simulink model "Platoon_Year1_CACC_fixed"  (R2026a)
settings: Solver=ode23tb  StopTime=inf  MaxStep=0.01  RelTol=1e-4  AbsTol=1e-6
values from neighbouring files (symbols this model uses):
  Cyber_AttackType = 0    [init_platoon_params.m]
  Cyber_FDI_Bias = 2    [init_platoon_params.m]
  Cyber_FDI_Field = 3    [init_platoon_params.m]
  Cyber_ReplayDelay = 0.5    [init_platoon_params.m]
  Cyber_ResidualThreshold = 1.0    (= 1)    [init_platoon_params.m]
  Cyber_TargetVehicle = 1    [init_platoon_params.m]
  D_DES = 10    [init_platoon_params.m]    (also in platoon_cyber_ui.m = evalin('base','D_DES'))
  h_CTH = 0.6    [init_platoon_params.m]
  Kd_CACC = 0.7    [init_platoon_params.m]
  Kd_PD = 0.10    (= 0.1)    [init_platoon_params.m]
  KP_CACC = 0.2    [init_platoon_params.m]
  Kp_PD = 0.8    [init_platoon_params.m]
  L_VEH = 4    [init_platoon_params.m]    (also in platoon_cyber_ui.m = evalin('base','L_VEH'))
  v0 = 0    [init_platoon_params.m]
  x0_f = x0_leader - (1:4) * gap0    [init_platoon_params.m]
  x0_leader = 130    [init_platoon_params.m]
undefined symbols (not defined in the file or in its folder): t_step
libraries: simulink x4
settings Model: Creator=robert  LastModifiedBy=Robert

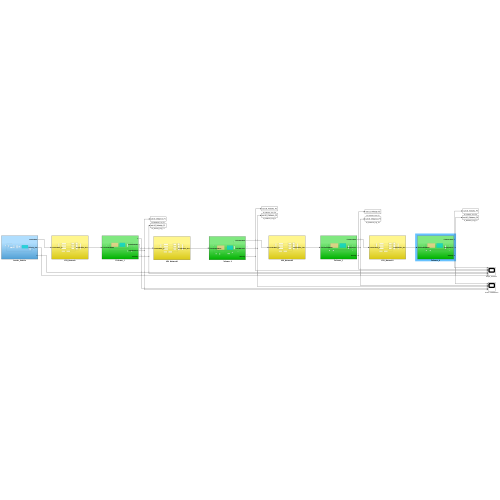
[thumbnail: Simulink's stored preview of the top-level diagram]
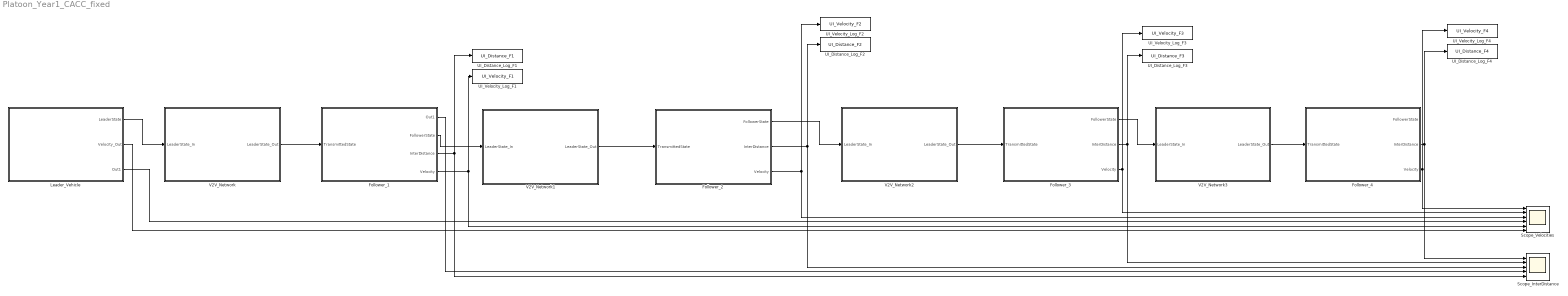
== system Platoon_Year1_CACC_fixed ==
  Follower_1 : Subsystem
  Follower_2 : Subsystem
  Follower_3 : Subsystem
  Follower_4 : Subsystem
  Leader_Vehicle : Subsystem
  Scope_InterDistance : Scope  NumInputPorts=5
      settings: ActiveDisplayYMinimum=-70.886144233669683  ActiveDisplayYMaximum=99.147830095673541
  Scope_Velocities : Scope  NumInputPorts=6
      settings: ActiveDisplayYMinimum=-4.6500669764690308  ActiveDisplayYMaximum=39.524777851018328
  UI_Distance_Log_F1 : ToWorkspace  VariableName=UI_Distance_F1  SaveFormat=Timeseries  SampleTime=-1
  UI_Distance_Log_F2 : ToWorkspace  VariableName=UI_Distance_F2  SaveFormat=Timeseries  SampleTime=-1
  UI_Distance_Log_F3 : ToWorkspace  VariableName=UI_Distance_F3  SaveFormat=Timeseries  SampleTime=-1
  UI_Distance_Log_F4 : ToWorkspace  VariableName=UI_Distance_F4  SaveFormat=Timeseries  SampleTime=-1
  UI_Velocity_Log_F1 : ToWorkspace  VariableName=UI_Velocity_F1  SaveFormat=Timeseries  SampleTime=-1
  UI_Velocity_Log_F2 : ToWorkspace  VariableName=UI_Velocity_F2  SaveFormat=Timeseries  SampleTime=-1
  UI_Velocity_Log_F3 : ToWorkspace  VariableName=UI_Velocity_F3  SaveFormat=Timeseries  SampleTime=-1
  UI_Velocity_Log_F4 : ToWorkspace  VariableName=UI_Velocity_F4  SaveFormat=Timeseries  SampleTime=-1
  V2V_Network : Subsystem
  V2V_Network1 : Subsystem
  V2V_Network2 : Subsystem
  V2V_Network3 : Subsystem
  wires:
  Follower_3/1(FollowerState) -> V2V_Network3/1(LeaderState_In)
  Follower_2/1(FollowerState) -> V2V_Network2/1(LeaderState_In)
  Follower_1/2(FollowerState) -> V2V_Network1/1(LeaderState_In)
  V2V_Network1/1(LeaderState_Out) -> Follower_2/1(TransmittedState)
  V2V_Network2/1(LeaderState_Out) -> Follower_3/1(TransmittedState)
  V2V_Network3/1(LeaderState_Out) -> Follower_4/1(TransmittedState)
  Leader_Vehicle/1(LeaderState) -> V2V_Network/1(LeaderState_In)
  V2V_Network/1(LeaderState_Out) -> Follower_1/1(TransmittedState)
  Leader_Vehicle/2(Velocity_Out) -> Scope_Velocities/6
  Follower_1/4(Velocity) -> Scope_Velocities/5, UI_Velocity_Log_F1/1
  Follower_2/3(Velocity) -> UI_Velocity_Log_F2/1, Scope_Velocities/3
  Follower_3/3(Velocity) -> Scope_Velocities/2, UI_Velocity_Log_F3/1
  Follower_4/3(Velocity) -> Scope_Velocities/1, UI_Velocity_Log_F4/1
  Follower_4/2(InterDistance) -> Scope_InterDistance/1, UI_Distance_Log_F4/1
  Follower_3/2(InterDistance) -> Scope_InterDistance/2, UI_Distance_Log_F3/1
  Follower_2/2(InterDistance) -> UI_Distance_Log_F2/1, Scope_InterDistance/3
  Follower_1/3(InterDistance) -> Scope_InterDistance/5, UI_Distance_Log_F1/1
  Follower_1/1(Out1) -> Scope_InterDistance/4
  Leader_Vehicle/3(Out1) -> Scope_Velocities/4

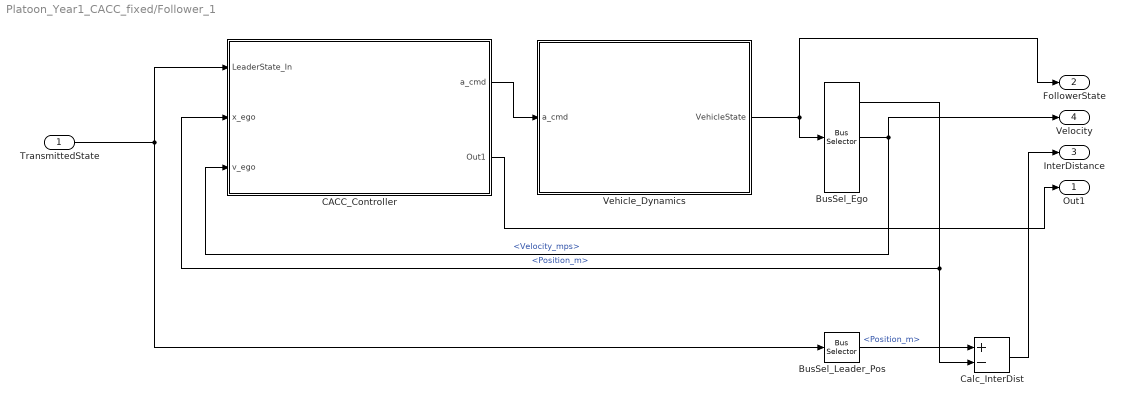
== system Platoon_Year1_CACC_fixed/Follower_1 ==
  TransmittedState : Inport
  BusSel_Ego : BusSelector  OutputSignals=Position_m,Velocity_mps,Accel_mps2
  BusSel_Leader_Pos : BusSelector  OutputSignals=Position_m
  CACC_Controller : Subsystem  TreatAsAtomicUnit=on
  Calc_InterDist : Sum  Inputs=+-
  Vehicle_Dynamics : Subsystem  TreatAsAtomicUnit=on
  Out1 : Outport
  FollowerState : Outport  Port=2
  InterDistance : Outport  Port=3
  Velocity : Outport  Port=4
  wires:
  TransmittedState/1 -> CACC_Controller/1(LeaderState_In), BusSel_Leader_Pos/1
  CACC_Controller/1(a_cmd) -> Vehicle_Dynamics/1(a_cmd)
  Vehicle_Dynamics/1(VehicleState) -> BusSel_Ego/1, FollowerState/1
  BusSel_Ego/1 -> CACC_Controller/2(x_ego), Calc_InterDist/2  "<Position_m>"
  BusSel_Ego/2 -> Velocity/1, CACC_Controller/3(v_ego)  "<Velocity_mps>"
  BusSel_Leader_Pos/1 -> Calc_InterDist/1  "<Position_m>"
  Calc_InterDist/1 -> InterDistance/1
  CACC_Controller/2(Out1) -> Out1/1

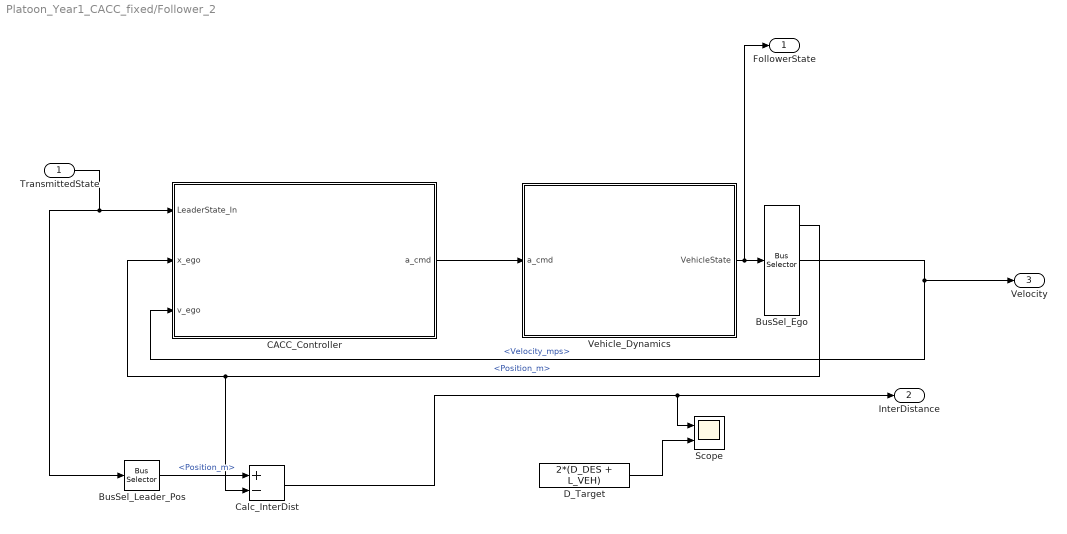
== system Platoon_Year1_CACC_fixed/Follower_2 ==
  TransmittedState : Inport
  BusSel_Ego : BusSelector  OutputSignals=Position_m,Velocity_mps,Accel_mps2
  BusSel_Leader_Pos : BusSelector  OutputSignals=Position_m
  CACC_Controller : Subsystem  TreatAsAtomicUnit=on
  Calc_InterDist : Sum  Inputs=+-
  D_Target : Constant  Value=2*(D_DES + L_VEH)
  Scope : Scope  NumInputPorts=2
      settings: ActiveDisplayYMinimum=-29.731224200783366  ActiveDisplayYMaximum=61.45407779195633
  Vehicle_Dynamics : Subsystem  TreatAsAtomicUnit=on
  FollowerState : Outport
  InterDistance : Outport  Port=2
  Velocity : Outport  Port=3
  wires:
  TransmittedState/1 -> CACC_Controller/1(LeaderState_In), BusSel_Leader_Pos/1
  CACC_Controller/1(a_cmd) -> Vehicle_Dynamics/1(a_cmd)
  Vehicle_Dynamics/1(VehicleState) -> BusSel_Ego/1, FollowerState/1
  BusSel_Ego/1 -> CACC_Controller/2(x_ego), Calc_InterDist/2  "<Position_m>"
  BusSel_Ego/2 -> CACC_Controller/3(v_ego), Velocity/1  "<Velocity_mps>"
  BusSel_Leader_Pos/1 -> Calc_InterDist/1  "<Position_m>"
  Calc_InterDist/1 -> InterDistance/1, Scope/1
  D_Target/1 -> Scope/2

== system Platoon_Year1_CACC_fixed/Follower_3 ==
  TransmittedState : Inport
  BusSel_Ego : BusSelector  OutputSignals=Position_m,Velocity_mps,Accel_mps2
  BusSel_Leader_Pos : BusSelector  OutputSignals=Position_m
  CACC_Controller : Subsystem  TreatAsAtomicUnit=on
  Calc_InterDist : Sum  Inputs=+-
  Vehicle_Dynamics : Subsystem  TreatAsAtomicUnit=on
  FollowerState : Outport
  InterDistance : Outport  Port=2
  Velocity : Outport  Port=3
  wires:
  TransmittedState/1 -> CACC_Controller/1(LeaderState_In), BusSel_Leader_Pos/1
  CACC_Controller/1(a_cmd) -> Vehicle_Dynamics/1(a_cmd)
  Vehicle_Dynamics/1(VehicleState) -> BusSel_Ego/1, FollowerState/1
  BusSel_Ego/1 -> CACC_Controller/2(x_ego), Calc_InterDist/2  "<Position_m>"
  BusSel_Ego/2 -> CACC_Controller/3(v_ego), Velocity/1  "<Velocity_mps>"
  BusSel_Leader_Pos/1 -> Calc_InterDist/1  "<Position_m>"
  Calc_InterDist/1 -> InterDistance/1

== system Platoon_Year1_CACC_fixed/Follower_4 ==
  TransmittedState : Inport
  BusSel_Ego : BusSelector  OutputSignals=Position_m,Velocity_mps,Accel_mps2
  BusSel_Leader_Pos : BusSelector  OutputSignals=Position_m
  CACC_Controller : Subsystem  TreatAsAtomicUnit=on
  Calc_InterDist : Sum  Inputs=+-
  Vehicle_Dynamics : Subsystem  TreatAsAtomicUnit=on
  FollowerState : Outport
  InterDistance : Outport  Port=2
  Velocity : Outport  Port=3
  wires:
  TransmittedState/1 -> CACC_Controller/1(LeaderState_In), BusSel_Leader_Pos/1
  CACC_Controller/1(a_cmd) -> Vehicle_Dynamics/1(a_cmd)
  Vehicle_Dynamics/1(VehicleState) -> BusSel_Ego/1, FollowerState/1
  BusSel_Ego/1 -> CACC_Controller/2(x_ego), Calc_InterDist/2  "<Position_m>"
  BusSel_Ego/2 -> CACC_Controller/3(v_ego), Velocity/1  "<Velocity_mps>"
  BusSel_Leader_Pos/1 -> Calc_InterDist/1  "<Position_m>"
  Calc_InterDist/1 -> InterDistance/1

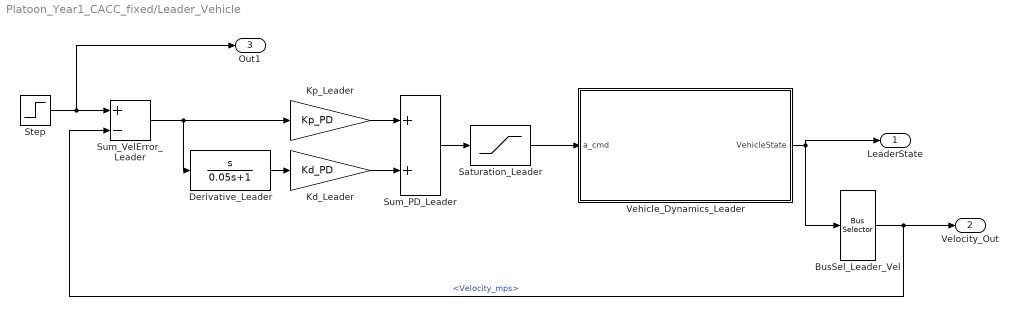
== system Platoon_Year1_CACC_fixed/Leader_Vehicle ==
  BusSel_Leader_Vel : BusSelector  OutputSignals=Velocity_mps
  Derivative_Leader : TransferFcn  Numerator=[1 0]  Denominator=[0.05 1]
  Kd_Leader : Gain  Gain=Kd_PD
  Kp_Leader : Gain  Gain=Kp_PD
  Saturation_Leader : Saturate  UpperLimit=2  LowerLimit=-4
  Step : Step  Time=t_step  InitialValue=v0  FinalValue=v_cmd_final  SampleTime=0.01
  Sum_PD_Leader : Sum
  Sum_VelError_Leader : Sum  Inputs=+-
  Vehicle_Dynamics_Leader : Subsystem  TreatAsAtomicUnit=on
  LeaderState : Outport
  Velocity_Out : Outport  Port=2
  Out1 : Outport  Port=3
  wires:
  Step/1 -> Out1/1, Sum_VelError_Leader/1
  Sum_VelError_Leader/1 -> Kp_Leader/1, Derivative_Leader/1
  Derivative_Leader/1 -> Kd_Leader/1
  Sum_PD_Leader/1 -> Saturation_Leader/1
  Saturation_Leader/1 -> Vehicle_Dynamics_Leader/1(a_cmd)
  Vehicle_Dynamics_Leader/1(VehicleState) -> LeaderState/1, BusSel_Leader_Vel/1
  BusSel_Leader_Vel/1 -> Sum_VelError_Leader/2, Velocity_Out/1  "<Velocity_mps>"
  Kd_Leader/1 -> Sum_PD_Leader/2
  Kp_Leader/1 -> Sum_PD_Leader/1

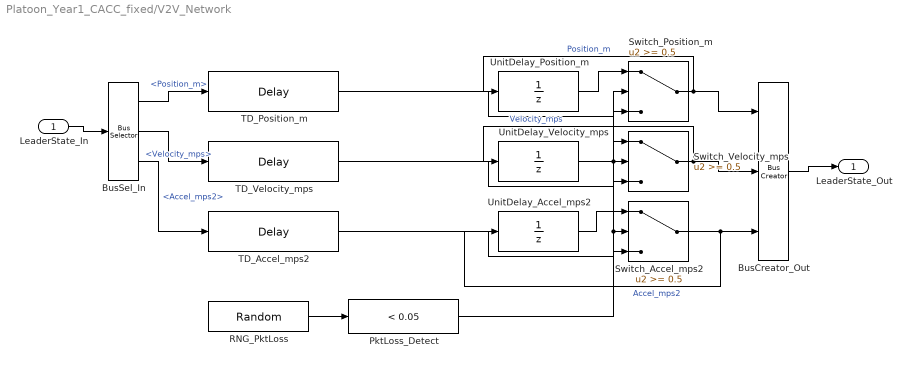
== system Platoon_Year1_CACC_fixed/V2V_Network ==
  LeaderState_In : Inport
  BusCreator_Out : BusCreator  Inputs=3
  BusSel_In : BusSelector  OutputSignals=Position_m,Velocity_mps,Accel_mps2
  PktLoss_Detect : simulink/Logic and Bit Operations/Compare To Constant  relop=<  const=0.05  OutDataTypeStr=boolean
  RNG_PktLoss : UniformRandomNumber  Minimum=0  Seed=42  SampleTime=0.01
  Switch_Accel_mps2 : Switch  Threshold=0.5  SaturateOnIntegerOverflow=off  InputSameDT=off
  Switch_Position_m : Switch  Threshold=0.5  SaturateOnIntegerOverflow=off  InputSameDT=off
  Switch_Velocity_mps : Switch  Threshold=0.5  SaturateOnIntegerOverflow=off  InputSameDT=off
  TD_Accel_mps2 : TransportDelay  DelayTime=0.02
  TD_Position_m : TransportDelay  DelayTime=0.02  InitialOutput=x0_leader
  TD_Velocity_mps : TransportDelay  DelayTime=0.02  InitialOutput=v0
  UnitDelay_Accel_mps2 : UnitDelay  SampleTime=0.01
  UnitDelay_Position_m : UnitDelay  InitialCondition=x0_leader  SampleTime=0.01
  UnitDelay_Velocity_mps : UnitDelay  InitialCondition=v0  SampleTime=0.01
  LeaderState_Out : Outport
  wires:
  BusSel_In/1 -> TD_Position_m/1  "<Position_m>"
  BusSel_In/2 -> TD_Velocity_mps/1  "<Velocity_mps>"
  BusSel_In/3 -> TD_Accel_mps2/1  "<Accel_mps2>"
  RNG_PktLoss/1 -> PktLoss_Detect/1
  UnitDelay_Position_m/1 -> Switch_Position_m/1
  PktLoss_Detect/1 -> Switch_Position_m/2, Switch_Velocity_mps/2, Switch_Accel_mps2/2
  TD_Position_m/1 -> Switch_Position_m/3
  Switch_Position_m/1 -> UnitDelay_Position_m/1, BusCreator_Out/1  "Position_m"
  UnitDelay_Velocity_mps/1 -> Switch_Velocity_mps/1
  TD_Velocity_mps/1 -> Switch_Velocity_mps/3
  Switch_Velocity_mps/1 -> UnitDelay_Velocity_mps/1, BusCreator_Out/2  "Velocity_mps"
  UnitDelay_Accel_mps2/1 -> Switch_Accel_mps2/1
  TD_Accel_mps2/1 -> Switch_Accel_mps2/3
  Switch_Accel_mps2/1 -> UnitDelay_Accel_mps2/1, BusCreator_Out/3  "Accel_mps2"
  BusCreator_Out/1 -> LeaderState_Out/1
  LeaderState_In/1 -> BusSel_In/1

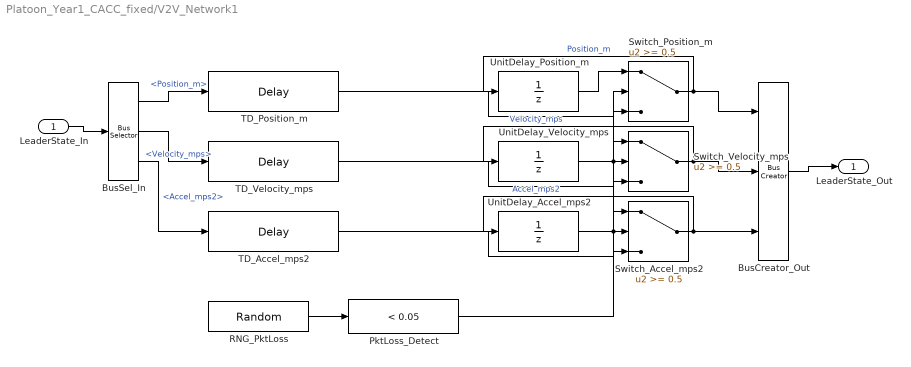
== system Platoon_Year1_CACC_fixed/V2V_Network1 ==
  LeaderState_In : Inport
  BusCreator_Out : BusCreator  Inputs=3
  BusSel_In : BusSelector  OutputSignals=Position_m,Velocity_mps,Accel_mps2
  PktLoss_Detect : simulink/Logic and Bit Operations/Compare To Constant  relop=<  const=0.05  OutDataTypeStr=boolean
  RNG_PktLoss : UniformRandomNumber  Minimum=0  Seed=137  SampleTime=0.01
  Switch_Accel_mps2 : Switch  Threshold=0.5  SaturateOnIntegerOverflow=off  InputSameDT=off
  Switch_Position_m : Switch  Threshold=0.5  SaturateOnIntegerOverflow=off  InputSameDT=off
  Switch_Velocity_mps : Switch  Threshold=0.5  SaturateOnIntegerOverflow=off  InputSameDT=off
  TD_Accel_mps2 : TransportDelay  DelayTime=0.02
  TD_Position_m : TransportDelay  DelayTime=0.02  InitialOutput=x0_f(1)
  TD_Velocity_mps : TransportDelay  DelayTime=0.02  InitialOutput=v0
  UnitDelay_Accel_mps2 : UnitDelay  SampleTime=0.01
  UnitDelay_Position_m : UnitDelay  InitialCondition=x0_f(1)  SampleTime=0.01
  UnitDelay_Velocity_mps : UnitDelay  InitialCondition=v0  SampleTime=0.01
  LeaderState_Out : Outport
  wires:
  BusSel_In/1 -> TD_Position_m/1  "<Position_m>"
  BusSel_In/2 -> TD_Velocity_mps/1  "<Velocity_mps>"
  BusSel_In/3 -> TD_Accel_mps2/1  "<Accel_mps2>"
  RNG_PktLoss/1 -> PktLoss_Detect/1
  UnitDelay_Position_m/1 -> Switch_Position_m/1
  PktLoss_Detect/1 -> Switch_Position_m/2, Switch_Velocity_mps/2, Switch_Accel_mps2/2
  TD_Position_m/1 -> Switch_Position_m/3
  Switch_Position_m/1 -> UnitDelay_Position_m/1, BusCreator_Out/1  "Position_m"
  UnitDelay_Velocity_mps/1 -> Switch_Velocity_mps/1
  TD_Velocity_mps/1 -> Switch_Velocity_mps/3
  Switch_Velocity_mps/1 -> UnitDelay_Velocity_mps/1, BusCreator_Out/2  "Velocity_mps"
  UnitDelay_Accel_mps2/1 -> Switch_Accel_mps2/1
  TD_Accel_mps2/1 -> Switch_Accel_mps2/3
  Switch_Accel_mps2/1 -> UnitDelay_Accel_mps2/1, BusCreator_Out/3  "Accel_mps2"
  BusCreator_Out/1 -> LeaderState_Out/1
  LeaderState_In/1 -> BusSel_In/1

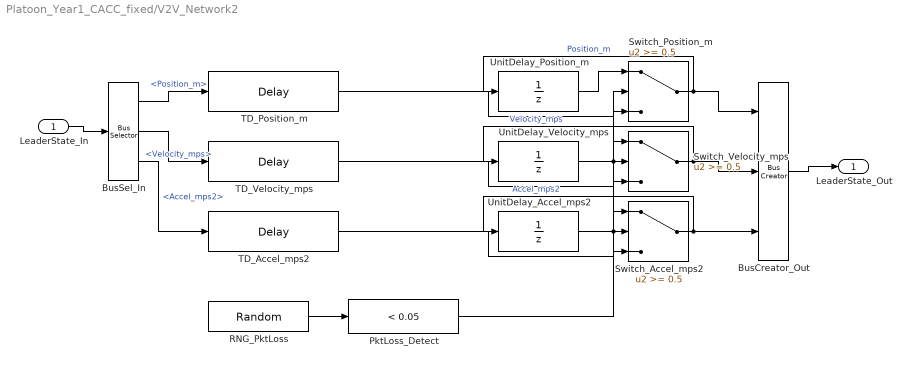
== system Platoon_Year1_CACC_fixed/V2V_Network2 ==
  LeaderState_In : Inport
  BusCreator_Out : BusCreator  Inputs=3
  BusSel_In : BusSelector  OutputSignals=Position_m,Velocity_mps,Accel_mps2
  PktLoss_Detect : simulink/Logic and Bit Operations/Compare To Constant  relop=<  const=0.05  OutDataTypeStr=boolean
  RNG_PktLoss : UniformRandomNumber  Minimum=0  Seed=251  SampleTime=0.01
  Switch_Accel_mps2 : Switch  Threshold=0.5  SaturateOnIntegerOverflow=off  InputSameDT=off
  Switch_Position_m : Switch  Threshold=0.5  SaturateOnIntegerOverflow=off  InputSameDT=off
  Switch_Velocity_mps : Switch  Threshold=0.5  SaturateOnIntegerOverflow=off  InputSameDT=off
  TD_Accel_mps2 : TransportDelay  DelayTime=0.02
  TD_Position_m : TransportDelay  DelayTime=0.02  InitialOutput=x0_f(2)
  TD_Velocity_mps : TransportDelay  DelayTime=0.02  InitialOutput=v0
  UnitDelay_Accel_mps2 : UnitDelay  SampleTime=0.01
  UnitDelay_Position_m : UnitDelay  InitialCondition=x0_f(2)  SampleTime=0.01
  UnitDelay_Velocity_mps : UnitDelay  InitialCondition=v0  SampleTime=0.01
  LeaderState_Out : Outport
  wires:
  BusSel_In/1 -> TD_Position_m/1  "<Position_m>"
  BusSel_In/2 -> TD_Velocity_mps/1  "<Velocity_mps>"
  BusSel_In/3 -> TD_Accel_mps2/1  "<Accel_mps2>"
  RNG_PktLoss/1 -> PktLoss_Detect/1
  UnitDelay_Position_m/1 -> Switch_Position_m/1
  PktLoss_Detect/1 -> Switch_Position_m/2, Switch_Velocity_mps/2, Switch_Accel_mps2/2
  TD_Position_m/1 -> Switch_Position_m/3
  Switch_Position_m/1 -> UnitDelay_Position_m/1, BusCreator_Out/1  "Position_m"
  UnitDelay_Velocity_mps/1 -> Switch_Velocity_mps/1
  TD_Velocity_mps/1 -> Switch_Velocity_mps/3
  Switch_Velocity_mps/1 -> UnitDelay_Velocity_mps/1, BusCreator_Out/2  "Velocity_mps"
  UnitDelay_Accel_mps2/1 -> Switch_Accel_mps2/1
  TD_Accel_mps2/1 -> Switch_Accel_mps2/3
  Switch_Accel_mps2/1 -> UnitDelay_Accel_mps2/1, BusCreator_Out/3  "Accel_mps2"
  BusCreator_Out/1 -> LeaderState_Out/1
  LeaderState_In/1 -> BusSel_In/1

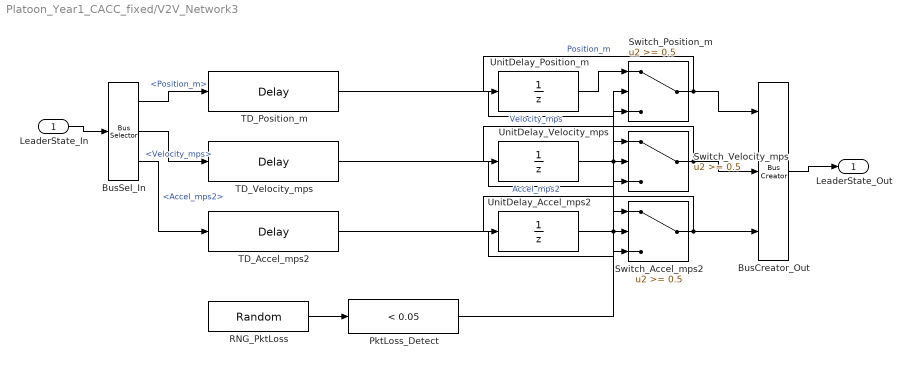
== system Platoon_Year1_CACC_fixed/V2V_Network3 ==
  LeaderState_In : Inport
  BusCreator_Out : BusCreator  Inputs=3
  BusSel_In : BusSelector  OutputSignals=Position_m,Velocity_mps,Accel_mps2
  PktLoss_Detect : simulink/Logic and Bit Operations/Compare To Constant  relop=<  const=0.05  OutDataTypeStr=boolean
  RNG_PktLoss : UniformRandomNumber  Minimum=0  Seed=389  SampleTime=0.01
  Switch_Accel_mps2 : Switch  Threshold=0.5  SaturateOnIntegerOverflow=off  InputSameDT=off
  Switch_Position_m : Switch  Threshold=0.5  SaturateOnIntegerOverflow=off  InputSameDT=off
  Switch_Velocity_mps : Switch  Threshold=0.5  SaturateOnIntegerOverflow=off  InputSameDT=off
  TD_Accel_mps2 : TransportDelay  DelayTime=0.02
  TD_Position_m : TransportDelay  DelayTime=0.02  InitialOutput=x0_f(3)
  TD_Velocity_mps : TransportDelay  DelayTime=0.02  InitialOutput=v0
  UnitDelay_Accel_mps2 : UnitDelay  SampleTime=0.01
  UnitDelay_Position_m : UnitDelay  InitialCondition=x0_f(3)  SampleTime=0.01
  UnitDelay_Velocity_mps : UnitDelay  InitialCondition=v0  SampleTime=0.01
  LeaderState_Out : Outport
  wires:
  BusSel_In/1 -> TD_Position_m/1  "<Position_m>"
  BusSel_In/2 -> TD_Velocity_mps/1  "<Velocity_mps>"
  BusSel_In/3 -> TD_Accel_mps2/1  "<Accel_mps2>"
  RNG_PktLoss/1 -> PktLoss_Detect/1
  UnitDelay_Position_m/1 -> Switch_Position_m/1
  PktLoss_Detect/1 -> Switch_Position_m/2, Switch_Velocity_mps/2, Switch_Accel_mps2/2
  TD_Position_m/1 -> Switch_Position_m/3
  Switch_Position_m/1 -> UnitDelay_Position_m/1, BusCreator_Out/1  "Position_m"
  UnitDelay_Velocity_mps/1 -> Switch_Velocity_mps/1
  TD_Velocity_mps/1 -> Switch_Velocity_mps/3
  Switch_Velocity_mps/1 -> UnitDelay_Velocity_mps/1, BusCreator_Out/2  "Velocity_mps"
  UnitDelay_Accel_mps2/1 -> Switch_Accel_mps2/1
  TD_Accel_mps2/1 -> Switch_Accel_mps2/3
  Switch_Accel_mps2/1 -> UnitDelay_Accel_mps2/1, BusCreator_Out/3  "Accel_mps2"
  BusCreator_Out/1 -> LeaderState_Out/1
  LeaderState_In/1 -> BusSel_In/1

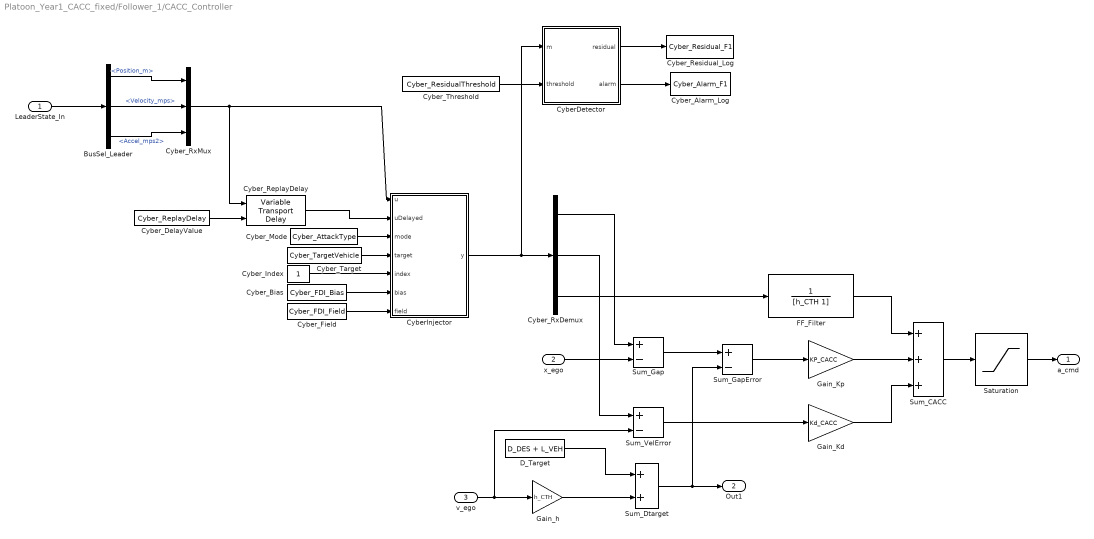
== system Platoon_Year1_CACC_fixed/Follower_1/CACC_Controller ==
  LeaderState_In : Inport
  x_ego : Inport  Port=2
  v_ego : Inport  Port=3
  BusSel_Leader : BusSelector  OutputSignals=Position_m,Velocity_mps,Accel_mps2
  CyberDetector : MATLAB Function  TreatAsAtomicUnit=on
  CyberInjector : MATLAB Function  TreatAsAtomicUnit=on
  Cyber_Alarm_Log : ToWorkspace  VariableName=Cyber_Alarm_F1  SaveFormat=Timeseries  SampleTime=-1
  Cyber_Bias : Constant  Value=Cyber_FDI_Bias
  Cyber_DelayValue : Constant  Value=Cyber_ReplayDelay
  Cyber_Field : Constant  Value=Cyber_FDI_Field
  Cyber_Index : Constant
  Cyber_Mode : Constant  Value=Cyber_AttackType
  Cyber_ReplayDelay : VariableTransportDelay  MaximumDelay=5  InitialOutput=[x0_leader; v0; 0]  MaximumPoints=8192
  Cyber_Residual_Log : ToWorkspace  VariableName=Cyber_Residual_F1  SaveFormat=Timeseries  SampleTime=-1
  Cyber_RxDemux : Demux  Outputs=3
  Cyber_RxMux : Mux  Inputs=3
  Cyber_Target : Constant  Value=Cyber_TargetVehicle
  Cyber_Threshold : Constant  Value=Cyber_ResidualThreshold
  D_Target : Constant  Value=D_DES + L_VEH
  FF_Filter : TransferFcn  Denominator=[h_CTH 1]
  Gain_Kd : Gain  Gain=Kd_CACC
  Gain_Kp : Gain  Gain=KP_CACC
  Gain_h : Gain  Gain=h_CTH
  Saturation : Saturate  UpperLimit=2  LowerLimit=-4
  Sum_CACC : Sum  Inputs=+++
  Sum_Dtarget : Sum
  Sum_Gap : Sum  Inputs=+-
  Sum_GapError : Sum  Inputs=+-
  Sum_VelError : Sum  Inputs=+-
  a_cmd : Outport
  Out1 : Outport  Port=2
  wires:
  BusSel_Leader/3 -> Cyber_RxMux/3  "<Accel_mps2>"
  CyberDetector/2(alarm) -> Cyber_Alarm_Log/1
  LeaderState_In/1 -> BusSel_Leader/1
  BusSel_Leader/1 -> Cyber_RxMux/1  "<Position_m>"
  Cyber_DelayValue/1 -> Cyber_ReplayDelay/2
  Cyber_RxMux/1 -> CyberInjector/1(u), Cyber_ReplayDelay/1
  Sum_GapError/1 -> Gain_Kp/1
  BusSel_Leader/2 -> Cyber_RxMux/2  "<Velocity_mps>"
  Sum_CACC/1 -> Saturation/1
  Cyber_ReplayDelay/1 -> CyberInjector/2(uDelayed)
  Cyber_Mode/1 -> CyberInjector/3(mode)
  Cyber_Target/1 -> CyberInjector/4(target)
  Gain_Kp/1 -> Sum_CACC/2
  Cyber_Index/1 -> CyberInjector/5(index)
  Cyber_Bias/1 -> CyberInjector/6(bias)
  Cyber_Field/1 -> CyberInjector/7(field)
  CyberInjector/1(y) -> Cyber_RxDemux/1, CyberDetector/1(m)
  Cyber_Threshold/1 -> CyberDetector/2(threshold)
  v_ego/1 -> Sum_VelError/2, Gain_h/1
  CyberDetector/1(residual) -> Cyber_Residual_Log/1
  Cyber_RxDemux/1 -> Sum_Gap/1
  Cyber_RxDemux/2 -> Sum_VelError/1
  Cyber_RxDemux/3 -> FF_Filter/1
  x_ego/1 -> Sum_Gap/2
  D_Target/1 -> Sum_Dtarget/1
  Gain_h/1 -> Sum_Dtarget/2
  Sum_Gap/1 -> Sum_GapError/1
  Sum_VelError/1 -> Gain_Kd/1
  Sum_Dtarget/1 -> Out1/1, Sum_GapError/2
  FF_Filter/1 -> Sum_CACC/1
  Gain_Kd/1 -> Sum_CACC/3
  Saturation/1 -> a_cmd/1

== system Platoon_Year1_CACC_fixed/Follower_1/Vehicle_Dynamics ==
  a_cmd : Inport
  BusCreator_VehState : BusCreator  Inputs=3
  Engine_Lag_TF : TransferFcn  Denominator=[0.15 1]
  Int_a2v : Integrator  InitialCondition=v0
  Int_v2x : Integrator  InitialCondition=104
  VehicleState : Outport
  wires:
  a_cmd/1 -> Engine_Lag_TF/1
  Engine_Lag_TF/1 -> Int_a2v/1, BusCreator_VehState/3  "Accel_mps2"
  Int_a2v/1 -> Int_v2x/1, BusCreator_VehState/2  "Velocity_mps"
  Int_v2x/1 -> BusCreator_VehState/1  "Position_m"
  BusCreator_VehState/1 -> VehicleState/1

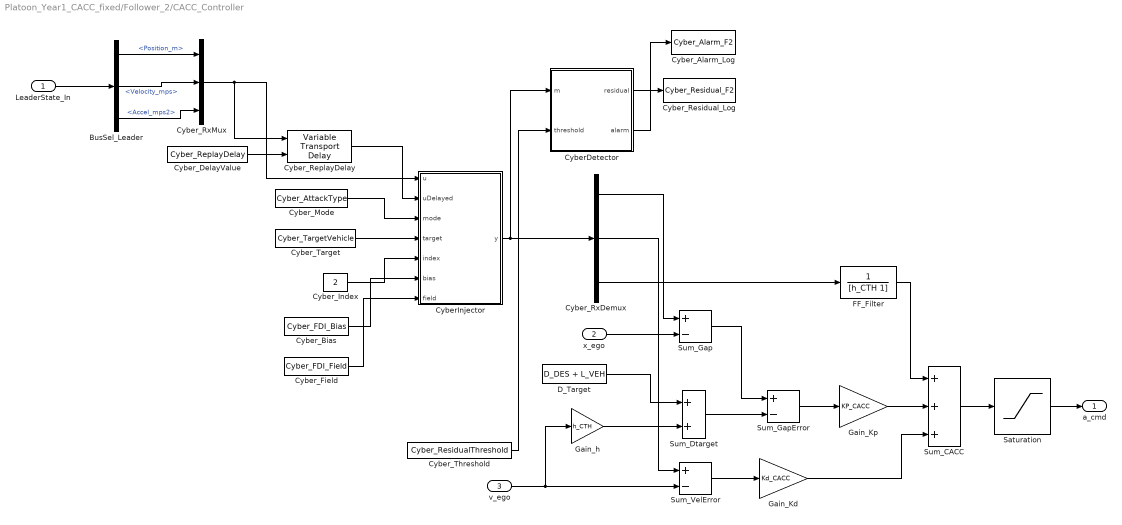
== system Platoon_Year1_CACC_fixed/Follower_2/CACC_Controller ==
  LeaderState_In : Inport
  x_ego : Inport  Port=2
  v_ego : Inport  Port=3
  BusSel_Leader : BusSelector  OutputSignals=Position_m,Velocity_mps,Accel_mps2
  CyberDetector : MATLAB Function  TreatAsAtomicUnit=on
  CyberInjector : MATLAB Function  TreatAsAtomicUnit=on
  Cyber_Alarm_Log : ToWorkspace  VariableName=Cyber_Alarm_F2  SaveFormat=Timeseries  SampleTime=-1
  Cyber_Bias : Constant  Value=Cyber_FDI_Bias
  Cyber_DelayValue : Constant  Value=Cyber_ReplayDelay
  Cyber_Field : Constant  Value=Cyber_FDI_Field
  Cyber_Index : Constant  Value=2
  Cyber_Mode : Constant  Value=Cyber_AttackType
  Cyber_ReplayDelay : VariableTransportDelay  MaximumDelay=5  InitialOutput=[x0_f(1); v0; 0]  MaximumPoints=8192
  Cyber_Residual_Log : ToWorkspace  VariableName=Cyber_Residual_F2  SaveFormat=Timeseries  SampleTime=-1
  Cyber_RxDemux : Demux  Outputs=3
  Cyber_RxMux : Mux  Inputs=3
  Cyber_Target : Constant  Value=Cyber_TargetVehicle
  Cyber_Threshold : Constant  Value=Cyber_ResidualThreshold
  D_Target : Constant  Value=D_DES + L_VEH
  FF_Filter : TransferFcn  Denominator=[h_CTH 1]
  Gain_Kd : Gain  Gain=Kd_CACC
  Gain_Kp : Gain  Gain=KP_CACC
  Gain_h : Gain  Gain=h_CTH
  Saturation : Saturate  UpperLimit=2  LowerLimit=-4
  Sum_CACC : Sum  Inputs=+++
  Sum_Dtarget : Sum
  Sum_Gap : Sum  Inputs=+-
  Sum_GapError : Sum  Inputs=+-
  Sum_VelError : Sum  Inputs=+-
  a_cmd : Outport
  wires:
  LeaderState_In/1 -> BusSel_Leader/1
  BusSel_Leader/2 -> Cyber_RxMux/2  "<Velocity_mps>"
  BusSel_Leader/1 -> Cyber_RxMux/1  "<Position_m>"
  BusSel_Leader/3 -> Cyber_RxMux/3  "<Accel_mps2>"
  FF_Filter/1 -> Sum_CACC/1
  Cyber_RxMux/1 -> CyberInjector/1(u), Cyber_ReplayDelay/1
  Cyber_Bias/1 -> CyberInjector/6(bias)
  Cyber_Mode/1 -> CyberInjector/3(mode)
  Cyber_RxDemux/2 -> Sum_VelError/1
  Cyber_DelayValue/1 -> Cyber_ReplayDelay/2
  Gain_Kp/1 -> Sum_CACC/2
  Cyber_ReplayDelay/1 -> CyberInjector/2(uDelayed)
  Cyber_Target/1 -> CyberInjector/4(target)
  Cyber_Index/1 -> CyberInjector/5(index)
  Cyber_Field/1 -> CyberInjector/7(field)
  x_ego/1 -> Sum_Gap/2
  CyberInjector/1(y) -> Cyber_RxDemux/1, CyberDetector/1(m)
  Cyber_Threshold/1 -> CyberDetector/2(threshold)
  v_ego/1 -> Sum_VelError/2, Gain_h/1
  CyberDetector/1(residual) -> Cyber_Residual_Log/1
  Gain_h/1 -> Sum_Dtarget/2
  CyberDetector/2(alarm) -> Cyber_Alarm_Log/1
  Cyber_RxDemux/1 -> Sum_Gap/1
  Cyber_RxDemux/3 -> FF_Filter/1
  D_Target/1 -> Sum_Dtarget/1
  Sum_VelError/1 -> Gain_Kd/1
  Sum_Gap/1 -> Sum_GapError/1
  Sum_Dtarget/1 -> Sum_GapError/2
  Sum_GapError/1 -> Gain_Kp/1
  Gain_Kd/1 -> Sum_CACC/3
  Sum_CACC/1 -> Saturation/1
  Saturation/1 -> a_cmd/1

== system Platoon_Year1_CACC_fixed/Follower_2/Vehicle_Dynamics ==
  a_cmd : Inport
  BusCreator_VehState : BusCreator  Inputs=3
  Engine_Lag_TF : TransferFcn  Denominator=[0.15 1]
  Int_a2v : Integrator  InitialCondition=v0
  Int_v2x : Integrator  InitialCondition=78
  VehicleState : Outport
  wires:
  a_cmd/1 -> Engine_Lag_TF/1
  Engine_Lag_TF/1 -> Int_a2v/1, BusCreator_VehState/3  "Accel_mps2"
  Int_a2v/1 -> Int_v2x/1, BusCreator_VehState/2  "Velocity_mps"
  Int_v2x/1 -> BusCreator_VehState/1  "Position_m"
  BusCreator_VehState/1 -> VehicleState/1

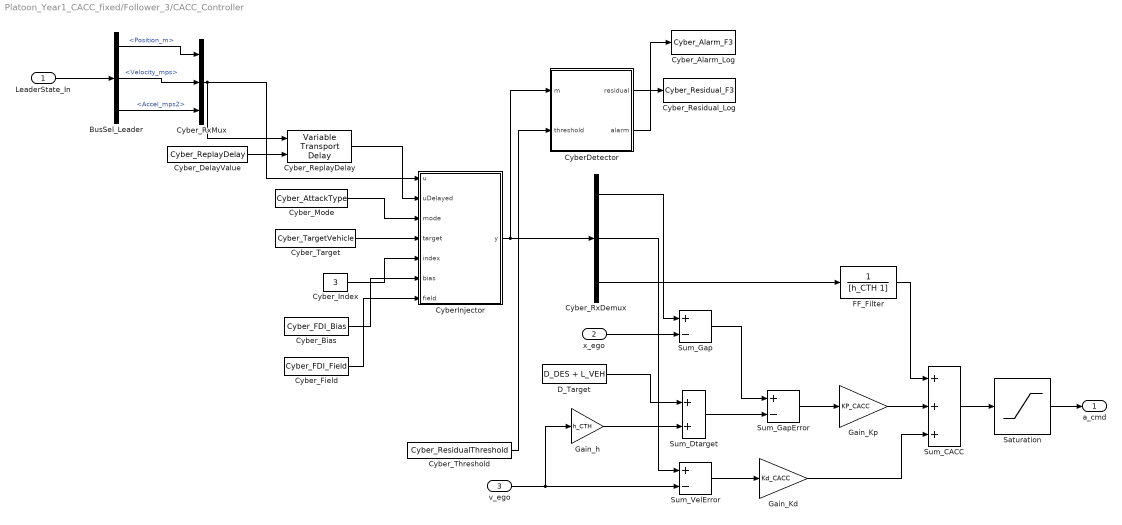
== system Platoon_Year1_CACC_fixed/Follower_3/CACC_Controller ==
  LeaderState_In : Inport
  x_ego : Inport  Port=2
  v_ego : Inport  Port=3
  BusSel_Leader : BusSelector  OutputSignals=Position_m,Velocity_mps,Accel_mps2
  CyberDetector : MATLAB Function  TreatAsAtomicUnit=on
  CyberInjector : MATLAB Function  TreatAsAtomicUnit=on
  Cyber_Alarm_Log : ToWorkspace  VariableName=Cyber_Alarm_F3  SaveFormat=Timeseries  SampleTime=-1
  Cyber_Bias : Constant  Value=Cyber_FDI_Bias
  Cyber_DelayValue : Constant  Value=Cyber_ReplayDelay
  Cyber_Field : Constant  Value=Cyber_FDI_Field
  Cyber_Index : Constant  Value=3
  Cyber_Mode : Constant  Value=Cyber_AttackType
  Cyber_ReplayDelay : VariableTransportDelay  MaximumDelay=5  InitialOutput=[x0_f(2); v0; 0]  MaximumPoints=8192
  Cyber_Residual_Log : ToWorkspace  VariableName=Cyber_Residual_F3  SaveFormat=Timeseries  SampleTime=-1
  Cyber_RxDemux : Demux  Outputs=3
  Cyber_RxMux : Mux  Inputs=3
  Cyber_Target : Constant  Value=Cyber_TargetVehicle
  Cyber_Threshold : Constant  Value=Cyber_ResidualThreshold
  D_Target : Constant  Value=D_DES + L_VEH
  FF_Filter : TransferFcn  Denominator=[h_CTH 1]
  Gain_Kd : Gain  Gain=Kd_CACC
  Gain_Kp : Gain  Gain=KP_CACC
  Gain_h : Gain  Gain=h_CTH
  Saturation : Saturate  UpperLimit=2  LowerLimit=-4
  Sum_CACC : Sum  Inputs=+++
  Sum_Dtarget : Sum
  Sum_Gap : Sum  Inputs=+-
  Sum_GapError : Sum  Inputs=+-
  Sum_VelError : Sum  Inputs=+-
  a_cmd : Outport
  wires:
  LeaderState_In/1 -> BusSel_Leader/1
  BusSel_Leader/2 -> Cyber_RxMux/2  "<Velocity_mps>"
  BusSel_Leader/1 -> Cyber_RxMux/1  "<Position_m>"
  Cyber_Mode/1 -> CyberInjector/3(mode)
  v_ego/1 -> Sum_VelError/2, Gain_h/1
  Cyber_RxMux/1 -> CyberInjector/1(u), Cyber_ReplayDelay/1
  BusSel_Leader/3 -> Cyber_RxMux/3  "<Accel_mps2>"
  Cyber_RxDemux/1 -> Sum_Gap/1
  Cyber_DelayValue/1 -> Cyber_ReplayDelay/2
  Cyber_ReplayDelay/1 -> CyberInjector/2(uDelayed)
  Cyber_Target/1 -> CyberInjector/4(target)
  Cyber_Index/1 -> CyberInjector/5(index)
  Cyber_Bias/1 -> CyberInjector/6(bias)
  Saturation/1 -> a_cmd/1
  Cyber_RxDemux/3 -> FF_Filter/1
  Cyber_Field/1 -> CyberInjector/7(field)
  CyberInjector/1(y) -> Cyber_RxDemux/1, CyberDetector/1(m)
  Gain_Kd/1 -> Sum_CACC/3
  Cyber_Threshold/1 -> CyberDetector/2(threshold)
  CyberDetector/1(residual) -> Cyber_Residual_Log/1
  CyberDetector/2(alarm) -> Cyber_Alarm_Log/1
  Cyber_RxDemux/2 -> Sum_VelError/1
  x_ego/1 -> Sum_Gap/2
  Sum_GapError/1 -> Gain_Kp/1
  Sum_Dtarget/1 -> Sum_GapError/2
  D_Target/1 -> Sum_Dtarget/1
  Gain_h/1 -> Sum_Dtarget/2
  Sum_VelError/1 -> Gain_Kd/1
  Sum_Gap/1 -> Sum_GapError/1
  FF_Filter/1 -> Sum_CACC/1
  Gain_Kp/1 -> Sum_CACC/2
  Sum_CACC/1 -> Saturation/1

== system Platoon_Year1_CACC_fixed/Follower_3/Vehicle_Dynamics ==
  a_cmd : Inport
  BusCreator_VehState : BusCreator  Inputs=3
  Engine_Lag_TF : TransferFcn  Denominator=[0.15 1]
  Int_a2v : Integrator  InitialCondition=v0
  Int_v2x : Integrator  InitialCondition=52
  VehicleState : Outport
  wires:
  a_cmd/1 -> Engine_Lag_TF/1
  Engine_Lag_TF/1 -> Int_a2v/1, BusCreator_VehState/3  "Accel_mps2"
  Int_a2v/1 -> Int_v2x/1, BusCreator_VehState/2  "Velocity_mps"
  Int_v2x/1 -> BusCreator_VehState/1  "Position_m"
  BusCreator_VehState/1 -> VehicleState/1

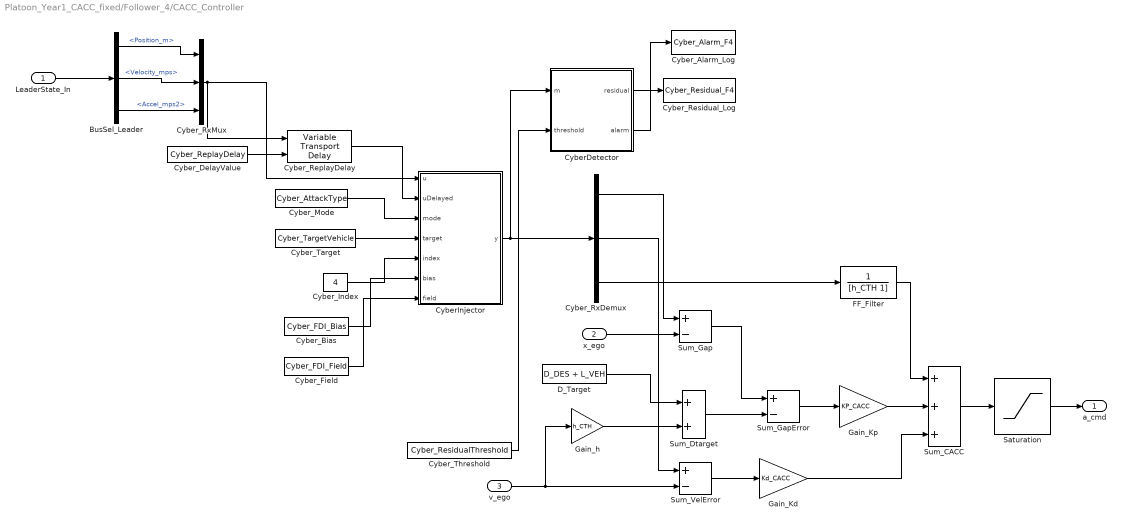
== system Platoon_Year1_CACC_fixed/Follower_4/CACC_Controller ==
  LeaderState_In : Inport
  x_ego : Inport  Port=2
  v_ego : Inport  Port=3
  BusSel_Leader : BusSelector  OutputSignals=Position_m,Velocity_mps,Accel_mps2
  CyberDetector : MATLAB Function  TreatAsAtomicUnit=on
  CyberInjector : MATLAB Function  TreatAsAtomicUnit=on
  Cyber_Alarm_Log : ToWorkspace  VariableName=Cyber_Alarm_F4  SaveFormat=Timeseries  SampleTime=-1
  Cyber_Bias : Constant  Value=Cyber_FDI_Bias
  Cyber_DelayValue : Constant  Value=Cyber_ReplayDelay
  Cyber_Field : Constant  Value=Cyber_FDI_Field
  Cyber_Index : Constant  Value=4
  Cyber_Mode : Constant  Value=Cyber_AttackType
  Cyber_ReplayDelay : VariableTransportDelay  MaximumDelay=5  InitialOutput=[x0_f(3); v0; 0]  MaximumPoints=8192
  Cyber_Residual_Log : ToWorkspace  VariableName=Cyber_Residual_F4  SaveFormat=Timeseries  SampleTime=-1
  Cyber_RxDemux : Demux  Outputs=3
  Cyber_RxMux : Mux  Inputs=3
  Cyber_Target : Constant  Value=Cyber_TargetVehicle
  Cyber_Threshold : Constant  Value=Cyber_ResidualThreshold
  D_Target : Constant  Value=D_DES + L_VEH
  FF_Filter : TransferFcn  Denominator=[h_CTH 1]
  Gain_Kd : Gain  Gain=Kd_CACC
  Gain_Kp : Gain  Gain=KP_CACC
  Gain_h : Gain  Gain=h_CTH
  Saturation : Saturate  UpperLimit=2  LowerLimit=-4
  Sum_CACC : Sum  Inputs=+++
  Sum_Dtarget : Sum
  Sum_Gap : Sum  Inputs=+-
  Sum_GapError : Sum  Inputs=+-
  Sum_VelError : Sum  Inputs=+-
  a_cmd : Outport
  wires:
  LeaderState_In/1 -> BusSel_Leader/1
  BusSel_Leader/2 -> Cyber_RxMux/2  "<Velocity_mps>"
  BusSel_Leader/3 -> Cyber_RxMux/3  "<Accel_mps2>"
  BusSel_Leader/1 -> Cyber_RxMux/1  "<Position_m>"
  Sum_CACC/1 -> Saturation/1
  Cyber_RxDemux/1 -> Sum_Gap/1
  Cyber_RxMux/1 -> CyberInjector/1(u), Cyber_ReplayDelay/1
  Cyber_DelayValue/1 -> Cyber_ReplayDelay/2
  Cyber_Mode/1 -> CyberInjector/3(mode)
  Cyber_ReplayDelay/1 -> CyberInjector/2(uDelayed)
  Sum_VelError/1 -> Gain_Kd/1
  Sum_Gap/1 -> Sum_GapError/1
  Cyber_RxDemux/2 -> Sum_VelError/1
  Cyber_Target/1 -> CyberInjector/4(target)
  Cyber_Index/1 -> CyberInjector/5(index)
  Cyber_Bias/1 -> CyberInjector/6(bias)
  Cyber_Field/1 -> CyberInjector/7(field)
  CyberInjector/1(y) -> Cyber_RxDemux/1, CyberDetector/1(m)
  Gain_Kd/1 -> Sum_CACC/3
  Cyber_Threshold/1 -> CyberDetector/2(threshold)
  v_ego/1 -> Sum_VelError/2, Gain_h/1
  CyberDetector/1(residual) -> Cyber_Residual_Log/1
  CyberDetector/2(alarm) -> Cyber_Alarm_Log/1
  Cyber_RxDemux/3 -> FF_Filter/1
  x_ego/1 -> Sum_Gap/2
  Sum_Dtarget/1 -> Sum_GapError/2
  D_Target/1 -> Sum_Dtarget/1
  Gain_h/1 -> Sum_Dtarget/2
  Sum_GapError/1 -> Gain_Kp/1
  FF_Filter/1 -> Sum_CACC/1
  Gain_Kp/1 -> Sum_CACC/2
  Saturation/1 -> a_cmd/1

== system Platoon_Year1_CACC_fixed/Follower_4/Vehicle_Dynamics ==
  a_cmd : Inport
  BusCreator_VehState : BusCreator  Inputs=3
  Engine_Lag_TF : TransferFcn  Denominator=[0.15 1]
  Int_a2v : Integrator  InitialCondition=v0
  Int_v2x : Integrator  InitialCondition=26
  VehicleState : Outport
  wires:
  a_cmd/1 -> Engine_Lag_TF/1
  Engine_Lag_TF/1 -> Int_a2v/1, BusCreator_VehState/3  "Accel_mps2"
  Int_a2v/1 -> Int_v2x/1, BusCreator_VehState/2  "Velocity_mps"
  Int_v2x/1 -> BusCreator_VehState/1  "Position_m"
  BusCreator_VehState/1 -> VehicleState/1

== system Platoon_Year1_CACC_fixed/Leader_Vehicle/Vehicle_Dynamics_Leader ==
  a_cmd : Inport
  BusCreator_VehState : BusCreator  Inputs=3
  Engine_Lag_TF : TransferFcn  Denominator=[0.15 1]
  Int_a2v : Integrator  InitialCondition=v0
  Int_v2x : Integrator  InitialCondition=130
  VehicleState : Outport
  wires:
  a_cmd/1 -> Engine_Lag_TF/1
  Engine_Lag_TF/1 -> Int_a2v/1, BusCreator_VehState/3  "Accel_mps2"
  Int_a2v/1 -> Int_v2x/1, BusCreator_VehState/2  "Velocity_mps"
  Int_v2x/1 -> BusCreator_VehState/1  "Position_m"
  BusCreator_VehState/1 -> VehicleState/1

== matlab function Platoon_Year1_CACC_fixed/Follower_2/CACC_Controller/CyberInjector ==
  settings: updateMethod=DISCRETE  sampleTime=0.01
  data: u input; y output; uDelayed input; mode input; target input; index input; bias input; field input
function y = cyber(u,uDelayed,mode,target,index,bias,field)
% Atac pe mesajul V2V al predecesorului, u = [x; v; a] (m, m/s, m/s^2).
persistent uLast
if isempty(uLast), uLast = u; end
y = u;
active = target == index;
isDoS = active && mode == 1;
if isDoS
    y = uLast; % DoS: mesaj blocat, receptorul pastreaza ultimul mesaj primit
elseif active && mode == 2
    k = min(max(round(field),1),3);
    y(k) = u(k) + bias; % FDI: bias aditiv pe campul ales (1 x, 2 v, 3 a)
elseif active && mode == 3
    y = uDelayed; % Replay: mesaj vechi retransmis
end
if ~isDoS, uLast = u; end
end

== matlab function Platoon_Year1_CACC_fixed/Follower_1/CACC_Controller/CyberInjector ==
  settings: updateMethod=DISCRETE  sampleTime=0.01
  data: u input; y output; uDelayed input; mode input; target input; index input; bias input; field input
function y = cyber(u,uDelayed,mode,target,index,bias,field)
% Atac pe mesajul V2V al predecesorului, u = [x; v; a] (m, m/s, m/s^2).
persistent uLast
if isempty(uLast), uLast = u; end
y = u;
active = target == index;
isDoS = active && mode == 1;
if isDoS
    y = uLast; % DoS: mesaj blocat, receptorul pastreaza ultimul mesaj primit
elseif active && mode == 2
    k = min(max(round(field),1),3);
    y(k) = u(k) + bias; % FDI: bias aditiv pe campul ales (1 x, 2 v, 3 a)
elseif active && mode == 3
    y = uDelayed; % Replay: mesaj vechi retransmis
end
if ~isDoS, uLast = u; end
end

== matlab function Platoon_Year1_CACC_fixed/Follower_3/CACC_Controller/CyberInjector ==
  settings: updateMethod=DISCRETE  sampleTime=0.01
  data: u input; y output; uDelayed input; mode input; target input; index input; bias input; field input
function y = cyber(u,uDelayed,mode,target,index,bias,field)
% Atac pe mesajul V2V al predecesorului, u = [x; v; a] (m, m/s, m/s^2).
persistent uLast
if isempty(uLast), uLast = u; end
y = u;
active = target == index;
isDoS = active && mode == 1;
if isDoS
    y = uLast; % DoS: mesaj blocat, receptorul pastreaza ultimul mesaj primit
elseif active && mode == 2
    k = min(max(round(field),1),3);
    y(k) = u(k) + bias; % FDI: bias aditiv pe campul ales (1 x, 2 v, 3 a)
elseif active && mode == 3
    y = uDelayed; % Replay: mesaj vechi retransmis
end
if ~isDoS, uLast = u; end
end

== matlab function Platoon_Year1_CACC_fixed/Follower_4/CACC_Controller/CyberInjector ==
  settings: updateMethod=DISCRETE  sampleTime=0.01
  data: u input; y output; uDelayed input; mode input; target input; index input; bias input; field input
function y = cyber(u,uDelayed,mode,target,index,bias,field)
% Atac pe mesajul V2V al predecesorului, u = [x; v; a] (m, m/s, m/s^2).
persistent uLast
if isempty(uLast), uLast = u; end
y = u;
active = target == index;
isDoS = active && mode == 1;
if isDoS
    y = uLast; % DoS: mesaj blocat, receptorul pastreaza ultimul mesaj primit
elseif active && mode == 2
    k = min(max(round(field),1),3);
    y(k) = u(k) + bias; % FDI: bias aditiv pe campul ales (1 x, 2 v, 3 a)
elseif active && mode == 3
    y = uDelayed; % Replay: mesaj vechi retransmis
end
if ~isDoS, uLast = u; end
end

== matlab function Platoon_Year1_CACC_fixed/Follower_1/CACC_Controller/CyberDetector ==
  settings: updateMethod=DISCRETE  sampleTime=0.01
  data: m input; residual output; threshold input; alarm output
function [residual,alarm] = detect(m,threshold)
% Plauzibilitate intre campurile mesajului primit m = [x; v; a]:
% d/dt(x) ~ v si d/dt(v) ~ a. Ambele parti trec prin acelasi filtru
% 1/(Tf s + 1), initializat cu primul mesaj (fara salt la pornire).
% Alarma doar daca reziduul depaseste pragul continuu 0.2 s (20 pasi de
% 0.01 s), ca pierderile izolate de pachete sa nu declanseze alarma.
% Primele 0.5 s detectorul doar se initializeaza (mesajul initial din
% intarzierea V2V este constant, deci neplauzibil la viteza nenula).
persistent prev f count n
Ts = 0.01; Tf = 0.1; k = Ts/(Tf + Ts);
if isempty(prev)
    prev = m; f = [m(2); m(2); m(3); m(3)]; count = 0; n = 0;
end
n = n + 1;
raw = [(m(1) - prev(1))/Ts; m(2); (m(2) - prev(2))/Ts; m(3)];
f = f + k*(raw - f);
prev = m;
residual = [abs(f(1) - f(2)); abs(f(3) - f(4))];
if n > 50 && max(residual) > threshold, count = count + 1; else, count = 0; end
alarm = count >= 20;
end

== matlab function Platoon_Year1_CACC_fixed/Follower_2/CACC_Controller/CyberDetector ==
  settings: updateMethod=DISCRETE  sampleTime=0.01
  data: m input; residual output; threshold input; alarm output
function [residual,alarm] = detect(m,threshold)
% Plauzibilitate intre campurile mesajului primit m = [x; v; a]:
% d/dt(x) ~ v si d/dt(v) ~ a. Ambele parti trec prin acelasi filtru
% 1/(Tf s + 1), initializat cu primul mesaj (fara salt la pornire).
% Alarma doar daca reziduul depaseste pragul continuu 0.2 s (20 pasi de
% 0.01 s), ca pierderile izolate de pachete sa nu declanseze alarma.
% Primele 0.5 s detectorul doar se initializeaza (mesajul initial din
% intarzierea V2V este constant, deci neplauzibil la viteza nenula).
persistent prev f count n
Ts = 0.01; Tf = 0.1; k = Ts/(Tf + Ts);
if isempty(prev)
    prev = m; f = [m(2); m(2); m(3); m(3)]; count = 0; n = 0;
end
n = n + 1;
raw = [(m(1) - prev(1))/Ts; m(2); (m(2) - prev(2))/Ts; m(3)];
f = f + k*(raw - f);
prev = m;
residual = [abs(f(1) - f(2)); abs(f(3) - f(4))];
if n > 50 && max(residual) > threshold, count = count + 1; else, count = 0; end
alarm = count >= 20;
end

== matlab function Platoon_Year1_CACC_fixed/Follower_3/CACC_Controller/CyberDetector ==
  settings: updateMethod=DISCRETE  sampleTime=0.01
  data: m input; residual output; threshold input; alarm output
function [residual,alarm] = detect(m,threshold)
% Plauzibilitate intre campurile mesajului primit m = [x; v; a]:
% d/dt(x) ~ v si d/dt(v) ~ a. Ambele parti trec prin acelasi filtru
% 1/(Tf s + 1), initializat cu primul mesaj (fara salt la pornire).
% Alarma doar daca reziduul depaseste pragul continuu 0.2 s (20 pasi de
% 0.01 s), ca pierderile izolate de pachete sa nu declanseze alarma.
% Primele 0.5 s detectorul doar se initializeaza (mesajul initial din
% intarzierea V2V este constant, deci neplauzibil la viteza nenula).
persistent prev f count n
Ts = 0.01; Tf = 0.1; k = Ts/(Tf + Ts);
if isempty(prev)
    prev = m; f = [m(2); m(2); m(3); m(3)]; count = 0; n = 0;
end
n = n + 1;
raw = [(m(1) - prev(1))/Ts; m(2); (m(2) - prev(2))/Ts; m(3)];
f = f + k*(raw - f);
prev = m;
residual = [abs(f(1) - f(2)); abs(f(3) - f(4))];
if n > 50 && max(residual) > threshold, count = count + 1; else, count = 0; end
alarm = count >= 20;
end

== matlab function Platoon_Year1_CACC_fixed/Follower_4/CACC_Controller/CyberDetector ==
  settings: updateMethod=DISCRETE  sampleTime=0.01
  data: m input; residual output; threshold input; alarm output
function [residual,alarm] = detect(m,threshold)
% Plauzibilitate intre campurile mesajului primit m = [x; v; a]:
% d/dt(x) ~ v si d/dt(v) ~ a. Ambele parti trec prin acelasi filtru
% 1/(Tf s + 1), initializat cu primul mesaj (fara salt la pornire).
% Alarma doar daca reziduul depaseste pragul continuu 0.2 s (20 pasi de
% 0.01 s), ca pierderile izolate de pachete sa nu declanseze alarma.
% Primele 0.5 s detectorul doar se initializeaza (mesajul initial din
% intarzierea V2V este constant, deci neplauzibil la viteza nenula).
persistent prev f count n
Ts = 0.01; Tf = 0.1; k = Ts/(Tf + Ts);
if isempty(prev)
    prev = m; f = [m(2); m(2); m(3); m(3)]; count = 0; n = 0;
end
n = n + 1;
raw = [(m(1) - prev(1))/Ts; m(2); (m(2) - prev(2))/Ts; m(3)];
f = f + k*(raw - f);
prev = m;
residual = [abs(f(1) - f(2)); abs(f(3) - f(4))];
if n > 50 && max(residual) > threshold, count = count + 1; else, count = 0; end
alarm = count >= 20;
end
